simulink model "SIMU_DIF_CBF_ponto_sensor_param"  (R2025b)
settings: Solver=VariableStepAuto  StartTime=0.0  StopTime=10.0  RelTol=1e-3
undefined symbols (not defined in the file): c, l, lambda, psc, rs, theta0, thg, x0, xg, xo, y0, yg, yo
settings Model: Creator=ADM  LastModifiedBy=Dell
settings DataIOCC: ReturnWorkspaceOutputs=off

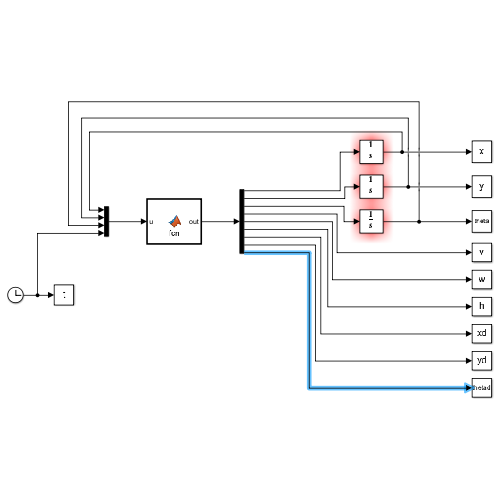
[thumbnail: Simulink's stored preview of the top-level diagram]
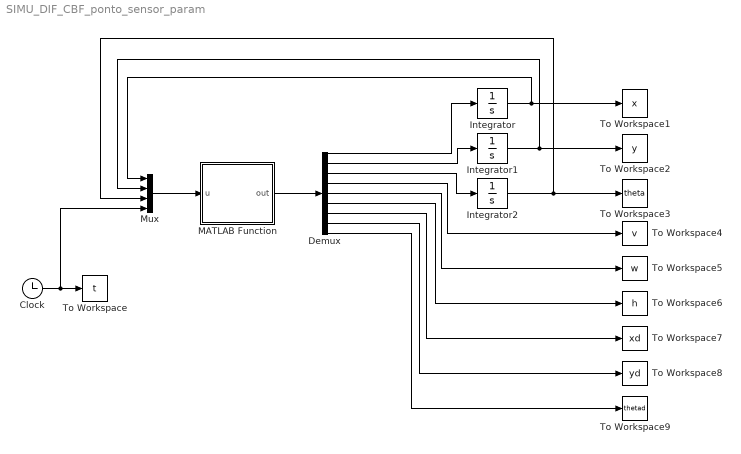
== system SIMU_DIF_CBF_ponto_sensor_param ==
  Clock : Clock
  Demux : Demux  Outputs=9
  Integrator : Integrator  InitialCondition=x0
  Integrator1 : Integrator  InitialCondition=y0
  Integrator2 : Integrator  InitialCondition=theta0
  MATLAB Function : MATLAB Function  TreatAsAtomicUnit=on
  Mux : Mux
  To Workspace : ToWorkspace  VariableName=t  SampleTime=-1
  To Workspace1 : ToWorkspace  VariableName=x  SampleTime=-1
  To Workspace2 : ToWorkspace  VariableName=y  SampleTime=-1
  To Workspace3 : ToWorkspace  VariableName=theta  SampleTime=-1
  To Workspace4 : ToWorkspace  VariableName=v  SampleTime=-1
  To Workspace5 : ToWorkspace  VariableName=w  SampleTime=-1
  To Workspace6 : ToWorkspace  VariableName=h  SampleTime=-1
  To Workspace7 : ToWorkspace  VariableName=xd  SampleTime=-1
  To Workspace8 : ToWorkspace  VariableName=yd  SampleTime=-1
  To Workspace9 : ToWorkspace  VariableName=thetad  SampleTime=-1
  wires:
  Clock/1 -> Mux/4, To Workspace/1
  Mux/1 -> MATLAB Function/1(u)
  MATLAB Function/1(out) -> Demux/1
  Demux/1 -> Integrator/1
  Demux/2 -> Integrator1/1
  Demux/3 -> Integrator2/1
  Integrator/1 -> To Workspace1/1, Mux/1
  Integrator1/1 -> To Workspace2/1, Mux/2
  Integrator2/1 -> To Workspace3/1, Mux/3
  Demux/4 -> To Workspace4/1
  Demux/5 -> To Workspace5/1
  Demux/6 -> To Workspace6/1
  Demux/7 -> To Workspace7/1
  Demux/8 -> To Workspace8/1
  Demux/9 -> To Workspace9/1

== matlab function SIMU_DIF_CBF_ponto_sensor_param/MATLAB Function ==
  data: u input size=4; out output size=9; xo parameter; yo parameter; l parameter; rs parameter; psc parameter; c parameter; lambda parameter; thg parameter; xg parameter; yg parameter
% https://chatgpt.com/c/6a83ac82-4ac8-83e9-bd58-c73133d80347
% tópico 3 - explica porque ficou pior com CLF + CBF
function out = fcn(u, xo, yo, xg, yg, thg, l, rs, psc, c, lambda)
x = u(1);
y = u(2);
theta = u(3);
t = u(4);

f_model = [0;0;0];
g_model = [cos(theta) 0;sin(theta) 0;0 1];

% % Atenção que nas referências lineares se o robô parar no centro do
% obtáculo, ele trava devido a dinâmica da CBF. Se jogar o obstáculo um pouco para baixo, ele escapa. Precisa estabeler uma
% lógica para ele escapar desta situação. Uma sugestão: forçar o robô ir para o lado ou virar.

% % Referência para pose
% xd = 5;
% yd = 5;
% thetad = pi/4;
% xd_dot = 0;
% yd_dot = 0;
% thetad_dot = 0;

% % Referência reta
% xd = 0.1*t;
% yd = 0;
% xd_dot = 0.1;
% yd_dot = 0;
% w_ref_const = 0;
% thetad = atan2(yd_dot, xd_dot);
% thetad_dot = w_ref_const;

% % Referência reta
% xd = 0.1*t;
% yd = 0.1*t;
% xd_dot = 0.1;
% yd_dot = 0.1;
% w_ref_const = 0;
% thetad = atan2(yd_dot, xd_dot);
% thetad_dot = w_ref_const;

% % % Referência de trajetória circular
% ===== OBSTACULOS (lidos do INIT) =====
obs  = [xo(:), yo(:)];
nobs = size(obs,1);

% ===== PONTO DE CHEGADA GUIADO POR "SENSOR" (sem trajetoria definida) =====
% A cada instante o robo usa sua propria pose, o ponto de chegada G e os obstaculos ao alcance.
% O alvo fica a Ld a frente, na direcao de G, deslocado lateralmente quando um obstaculo
% bloqueia o caminho direto (lado de MENOR desvio; exatamente sobre a linha: pela direita).
G    = [xg; yg];  thG = thg;    % ponto e orientacao de chegada (parametros xg, yg, thg do INIT)
m    = 0.05;    % folga alem de rs
pw   = 1.2;     % meia-largura da deformacao [m]
Ld   = 0.6;     % distancia do alvo a frente do robo [m]
Lb   = 1.5;     % distancia de G a partir da qual a orientacao final passa a contar [m]
Rsen = 3.0;     % alcance do sensor de obstaculos [m]
Lrot = 0.005;   % distancia de G a partir da qual o robo gira no lugar ate thG [m] (5 mm)
cm   = rs + m;
gx = G(1) - x;  gy = G(2) - y;
Lg = sqrt(gx^2 + gy^2);
if Lg > 1e-6
    ur = [gx; gy]/Lg;
else
    ur = [cos(theta); sin(theta)];
end
nr = [-ur(2); ur(1)];
angG = atan2(ur(2), ur(1));
st = min(Lg, Ld);
l0 = 0;  l1 = 0;
for i = 1:nobs
    so   = (obs(i,1)-x)*ur(1) + (obs(i,2)-y)*ur(2);
    dlat = (obs(i,1)-x)*nr(1) + (obs(i,2)-y)*nr(2);
    if so > -0.3 && so < min(Rsen, Lg + 0.3) && abs(dlat) < cm   % so obstaculos ao alcance e antes de G
        if abs(dlat) < 1e-3
            ell = -cm;
        else
            ell = dlat - sign(dlat)*cm;
        end
        sg = (st - so)/pw;
        if abs(sg) < 1
            l0 = l0 + ell*0.5*(1 + cos(pi*sg));
            l1 = l1 - ell*0.5*sin(pi*sg)*pi/pw;
        end
    end
end
xd = x + st*ur(1) + l0*nr(1);           % alvo
yd = y + st*ur(2) + l0*nr(2);
tht  = angG + atan(l1);                 % orientacao tangente ao desvio
lamb = min(max(1 - Lg/Lb, 0), 1);       % 0 longe de G, 1 ao chegar
thetad = tht + lamb*atan2(sin(thG - tht), cos(thG - tht));
xd_dot = 0;  yd_dot = 0;  thetad_dot = 0;

% % CLF + CBF - Vale para pose e trajetória
% % Primeira sugestão para V
% V = ((xd-x)^2 + (yd-y)^2 + (wrapToPi(thetad-theta))^2)/2;
% %V = ((xd-x)^2 + (yd-y)^2 + (thetad-theta)^2)/2;
% %V = ((x-xd)^2 + (y-yd)^2 + (theta-thetad)^2)/2;
% LfV = 0;
% LgV = [cos(theta)*(x - xd) + sin(theta)*(y - yd), wrapToPi(theta - thetad)];
% %LgV = [cos(theta)*(x - xd) + sin(theta)*(y - yd), theta - thetad];
% Vt = - thetad_dot*(wrapToPi(theta - thetad)) - xd_dot*(x - xd) - yd_dot*(y - yd);
% %Vt = - thetad_dot*(theta - thetad) - xd_dot*(x - xd) - yd_dot*(y - yd);

% % Teoricamente o mesmo resultado da CLF anterior - Só muda que não foram
% feitas as siplificações
% ex = cos(theta)*(xd-x) + sin(theta)*(yd-y);
% ey = -sin(theta)*(xd-x) + cos(theta)*(yd-y);
% etheta = wrapToPi(thetad-theta);
% % ex = cos(theta)*(x-xd) + sin(theta)*(y-yd);
% % ey = -sin(theta)*(x-xd) + cos(theta)*(y-yd);
% % etheta = wrapToPi(theta-thetad);
% V = ((ex)^2 + (ey)^2 + (etheta)^2)/2;
% % V = (wrapToPi(theta - thetad))^2/2 + (cos(theta)*(x - xd) + sin(theta)*(y - yd))^2/2 + (cos(theta)*(y - yd) - sin(theta)*(x - xd))^2/2;
% % V = (theta - thetad)^2/2 + (cos(theta)*(x - xd) + sin(theta)*(y - yd))^2/2 + (cos(theta)*(y - yd) - sin(theta)*(x - xd))^2/2;
% LfV = 0;
% %LfV = 0;
% %LgV = [cos(theta)*(cos(theta)*(cos(theta)*(x - xd) + sin(theta)*(y - yd)) - sin(theta)*(cos(theta)*(y - yd) - sin(theta)*(x - xd))) + sin(theta)*(cos(theta)*(cos(theta)*(y - yd) - sin(theta)*(x - xd)) + sin(theta)*(cos(theta)*(x - xd) + sin(theta)*(y - yd))), theta - thetad];
% %LgV = [cos(theta)*(cos(theta)*(cos(theta)*(x - xd) + sin(theta)*(y - yd)) - sin(theta)*(cos(theta)*(y - yd) - sin(theta)*(x - xd))) + sin(theta)*(cos(theta)*(cos(theta)*(y - yd) - sin(theta)*(x - xd)) + sin(theta)*(cos(theta)*(x - xd) + sin(theta)*(y - yd))), theta - thetad];
% LgV = [x*cos(theta) - xd*cos(theta) + y*sin(theta) - yd*sin(theta), wrapToPi(theta - thetad)];
% %LgV = [x*cos(theta) - xd*cos(theta) + y*sin(theta) - yd*sin(theta), theta - thetad];
% % Resposta Chatgpt
% %LgV = [cos(theta)*(x-xd) + sin(theta)*(y-yd), theta-thetad];
% % https://chatgpt.com/c/6a83ac82-4ac8-83e9-bd58-c73133d80347
% % tópico 5 e 6 explica porque usar este Vt
% %Vt = - xd_dot*(cos(theta)*(cos(theta)*(x - xd) + sin(theta)*(y - yd)) - sin(theta)*(cos(theta)*(y - yd) - sin(theta)*(x - xd))) - yd_dot*(cos(theta)*(cos(theta)*(y - yd) - sin(theta)*(x - xd)) + sin(theta)*(cos(theta)*(x - xd) + sin(theta)*(y - yd))) - thetad_dot*(theta - thetad);
% %Vt = - xd_dot*(cos(theta)*(cos(theta)*(x - xd) + sin(theta)*(y - yd)) - sin(theta)*(cos(theta)*(y - yd) - sin(theta)*(x - xd))) - yd_dot*(cos(theta)*(cos(theta)*(y - yd) - sin(theta)*(x - xd)) + sin(theta)*(cos(theta)*(x - xd) + sin(theta)*(y - yd))) - thetad_dot*(theta - thetad);
% %Vt = thetad*thetad_dot - theta*thetad_dot - x*xd_dot + xd*xd_dot - y*yd_dot + yd*yd_dot;
% %Vt = thetad*thetad_dot - theta*thetad_dot - x*xd_dot + xd*xd_dot - y*yd_dot + yd*yd_dot;
% Vt = - thetad_dot*(wrapToPi(theta - thetad)) - xd_dot*(x - xd) - yd_dot*(y - yd);

% % Outra sugestão de V - Resultados próximos
% % https://chatgpt.com/c/6ab10b65-7680-83e9-af95-79e091eac54d - explicação
% % a favor desta CLF - se for usar esta CLF, preciso descobrir de qual
% % referência o chatgpt tirou esta CLF
ex = cos(theta)*(xd-x) + sin(theta)*(yd-y);
ey = -sin(theta)*(xd-x) + cos(theta)*(yd-y);
etheta = thetad-theta;
%etheta = wrapToPi(thetad-theta);
ctheta = 1;
V = ((ex)^2 + (ey)^2)/2 + ctheta*(1-cos(etheta));
LfV = 0;
% LgV = [cos(theta)*(cos(theta)*(cos(theta)*(x - xd) + sin(theta)*(y - yd)) - sin(theta)*(cos(theta)*(y - yd) - sin(theta)*(x - xd))) + sin(theta)*(cos(theta)*(cos(theta)*(y - yd) - sin(theta)*(x - xd)) + sin(theta)*(cos(theta)*(x - xd) + sin(theta)*(y - yd))), ctheta*sin(theta - thetad)];
LgV = [x*cos(theta) - xd*cos(theta) + y*sin(theta) - yd*sin(theta), ctheta*sin(theta - thetad)];
% Vt = - xd_dot*(cos(theta)*(cos(theta)*(x - xd) + sin(theta)*(y - yd)) - sin(theta)*(cos(theta)*(y - yd) - sin(theta)*(x - xd))) - yd_dot*(cos(theta)*(cos(theta)*(y - yd) - sin(theta)*(x - xd)) + sin(theta)*(cos(theta)*(x - xd) + sin(theta)*(y - yd))) - ctheta*thetad_dot*sin(theta - thetad);
Vt = xd*xd_dot - x*xd_dot - y*yd_dot + yd*yd_dot - ctheta*thetad_dot*sin(theta - thetad);

% % CBF
% ===== OBSTACULOS (CBF individual + vies de lado) =====
% ===== OBSTACULOS: vetores xo, yo vindos do INIT (um elemento por obstaculo) =====
side = 1;      % +1 desvia virando a esquerda, -1 a direita
hact = 1.0;    % h abaixo do qual o vies de lado comeca
wb   = 0.0;    % intensidade maxima do vies em w [rad/s]

px = x + l*cos(theta);
py = y + l*sin(theta);

hv    = zeros(nobs,1);
Lghm  = zeros(nobs,2);
wbias = 0;
for i = 1:nobs
    dx = px - obs(i,1);
    dy = py - obs(i,2);
    hv(i)     = dx^2 + dy^2 - rs^2;
    Lghm(i,:) = [2*dx*cos(theta) + 2*dy*sin(theta), ...
                 2*l*(dy*cos(theta) - dx*sin(theta))];
    dist  = max(sqrt(dx^2 + dy^2), 1e-6);
    a     = max(0, min(1, 1 - hv(i)/hact));
    ahead = max(0, (-dx*cos(theta) - dy*sin(theta))/dist);
    wbias = wbias + side*a*ahead;
end
wbias = wb*max(-1, min(1, wbias));

h   = min(hv);   % apenas para o grafico
Lfh = 0;

% ===== CONTROLE NOMINAL DE RASTREAMENTO (Kanayama) =====
kp = 0.8;  ka = 2.0;  kb = -0.5;  krot = 2.0;   % controlador polar (kp>0, kb<0, ka>kp)
rho = sqrt((xd-x)^2 + (yd-y)^2);
al  = atan2(yd-y, xd-x) - theta;
al  = atan2(sin(al), cos(al));
be  = thetad - theta - al;
be  = atan2(sin(be), cos(be));
v_nom = kp*rho*max(cos(al), 0);         % nao anda de re: vira antes de avancar
w_nom = ka*al + kb*lamb*be + wbias;
if Lg < Lrot                            % chegou: gira no lugar ate a orientacao final
    v_nom = 0;
    w_nom = krot*atan2(sin(thG - theta), cos(thG - theta));
end
u_nom = [v_nom; w_nom];

% QP: minimiza ||u - u_nom||^2 + psc*delta^2
Hqp = [1 0 0; 0 1 0; 0 0 psc];
Fqp = [-u_nom; 0];

% ===== RESTRICOES: 1 CLF + nobs CBFs + limites de v e w =====
Aqp = zeros(nobs+5,3);
bqp = zeros(nobs+5,1);
Aqp(1,:) = [LgV, -1];
bqp(1)   = -LfV - c*V - Vt;
for i = 1:nobs
    Aqp(1+i,:) = [-Lghm(i,:), 0];
    bqp(1+i)   = Lfh + lambda*hv(i);
end
Aqp(nobs+2:nobs+5,:) = [1 0 0; -1 0 0; 0 1 0; 0 -1 0];
bqp(nobs+2:nobs+5)   = 2;

ucont = [0;0;0];
coder.extrinsic('QPhild');
ucont = QPhild(Hqp,Fqp,Aqp,bqp);
uc = [ucont(1,1);ucont(2,1)];
xmponto = f_model + g_model*uc;

% Saidas de referencia para o grafico: CIRCULO ORIGINAL (sem deformacao).
% O controle usa internamente a referencia deformada (xd, yd, thetad).
% Saidas de referencia para o grafico: ponto de chegada.
xd0 = G(1);
yd0 = G(2);
thetad0 = thG;
out = [xmponto(1,1);xmponto(2,1);xmponto(3,1);uc(1,1);uc(2,1);h;xd0;yd0;thetad0];








% % % Controle nominal + CBF - Safety Filter
% function out = fcn(u, xo, yo, l, rs, psc, c, lambda)
% x = u(1);
% y = u(2);
% theta = u(3);
% t = u(4);
% 
% f_model = [0;0;0];
% g_model = [cos(theta) 0;sin(theta) 0;0 1];
% 
% % % % Atenção que nas referências lineares se o robô parar no centro do
% % % obtáculo, ele trava devido a dinâmica da CBF. Se jogar o obstáculo um pouco para baixo, ele escapa 
% % % (Para o controle nominal, precisa jogar mais para baixo ainda). Precisa estabeler uma
% % % lógica para ele escapar desta situação. Uma sugestão: forçar o robô ir para o lado ou virar.
% 
% % % % Referência reta
% % xd = 0.1*t;
% % yd = 0;
% % xd_dot = 0.1;
% % yd_dot = 0;
% % w_ref_const = 0;
% % vd = sqrt(xd_dot^2 + yd_dot^2);
% % thetad = atan2(yd_dot, xd_dot);
% % wd = w_ref_const;
% 
% % % % Referência reta
% % xd = 0.1*t;
% % yd = 0.1*t;
% % xd_dot = 0.1;
% % yd_dot = 0.1;
% % w_ref_const = 0;
% % vd = sqrt(xd_dot^2 + yd_dot^2);
% % thetad = atan2(yd_dot, xd_dot);
% % wd = w_ref_const;
% 
% % % % Referência de trajetória circular
% % R = 2;
% % w_ref_const = 0.25;
% % xd = R*cos(w_ref_const*t);
% % yd = R*sin(w_ref_const*t);
% % xd_dot = -R*w_ref_const*sin(w_ref_const*t);
% % yd_dot =  R*w_ref_const*cos(w_ref_const*t);
% % vd = sqrt(xd_dot^2 + yd_dot^2);
% % thetad = atan2(yd_dot, xd_dot);
% % wd = w_ref_const;
% 
% % % % Controlador nominal para trajetória
% % kx = 1.5;
% % ky = 3.0;
% % ktheta = 2.0;
% % ex = cos(theta)*(xd-x) + sin(theta)*(yd-y);
% % ey = -sin(theta)*(xd-x) + cos(theta)*(yd-y);
% % %etheta = thetad-theta;
% % etheta = wrapToPi(thetad-theta);
% % % % https://chatgpt.com/c/6a83ac82-4ac8-83e9-bd58-c73133d80347 - nos
% % % % tópicos finais explica que com ky*vd*ey é melhor - nas simulações também
% % unom = [vd*cos(etheta)+kx*ex;wd+ky*vd*ey+ktheta*sin(etheta)];
% % %unom = [vd*cos(etheta)+kx*ex;wd+ky*ey+ktheta*sin(etheta)];
% 
% % % % Referência para pose
% xd = 5;
% yd = 5;
% thetad = pi/4;
% xd_dot = 0;
% yd_dot = 0;
% thetad_dot = 0;
% 
% % % % Controlador nominal para pose
% ex = xd - x;
% ey = yd - y;
% pho = sqrt(ex^2 + ey^2);
% alfa = atan2(ey,ex) - theta;
% % % wrapToPi e atan2 tem a mesma função: garantir que o ângulo fique entre
% % -pi e + pi
% %alfa = atan2(sin(alfa),cos(alfa));
% alfa = wrapToPi(alfa);
% % testar com estas duas possibilidades para beta
% %beta = thetad - theta;
% beta = thetad - theta - alfa;
% % % wrapToPi e atan2 tem a mesma função: garantir que o ângulo fique entre
% % -pi e + pi
% beta = wrapToPi(beta);
% % beta = atan2(sin(beta),cos(beta));
% kpho = 0.5;
% kalfa = 2;
% %kbeta = 0.5;
% kbeta = -0.5;
% % Tem duas opções de controle:
% % a princípio os resultados são parecidos, mas a primeira opção é melhor
% unom = [kpho*pho*cos(alfa);kalfa*alfa + kbeta*beta];
% % kv = 0.5;
% % kw = 1.0;
% % unom = [kv*pho;kw*alfa];
% 
% % ex = cos(theta)*(xd-x) + sin(theta)*(yd-y);
% % ey = -sin(theta)*(xd-x) + cos(theta)*(yd-y);
% % etheta = thetad-theta;
% % etheta = atan2(sin(etheta),cos(etheta));
% % kx = 5;
% % ky = 5;
% % ktheta = 5;
% % unom = [kx*ex;ky*ey + ktheta*etheta];
% 
% % % CBF
% h = (x+l*cos(theta)-xo)^2 + (y+l*sin(theta)-yo)^2 - (rs)^2;
% Lfh = 0;
% Lgh = [sin(theta)*(2*y - 2*yo + 2*l*sin(theta)) + cos(theta)*(2*x - 2*xo + 2*l*cos(theta)), 2*l*cos(theta)*(y - yo + l*sin(theta)) - 2*l*sin(theta)*(x - xo + l*cos(theta))];
% %Lgh = [sin(theta)*(2*y - 2*yo + 2*l*sin(theta)) + cos(theta)*(2*x - 2*xo + 2*l*cos(theta)), 2*l*cos(theta)*(y - yo + l*sin(theta)) - 2*l*sin(theta)*(x - xo + l*cos(theta))];
% 
% % % Controlador Final
% Hqp = [2];
% Fqp = [-2*unom];
% % Aqp = [-Lgh];
% % bqp = [Lfh+lambda*h];
% Aqp = [-Lgh;1 0;-1 0;0 1;0 -1];
% bqp = [Lfh+lambda*h;0.5;0.5;1.5;1.5];
% uc = [0;0];
% coder.extrinsic('QPhild');
% uc = QPhild(Hqp,Fqp,Aqp,bqp);
% xmponto = f_model + g_model*uc;
% %xmponto = f_model + g_model*unom;
% 
% % % Soluções Fechadas
% % % Não sei porque esta solução não funciona para este problema
% % %uc = [0;0];
% % I = Lfh + Lgh*unom;
% % J = lambda*h;
% % if (I<J)
% % ucont = -((I-J)/(norm(Lgh))^2)*(transpose(Lgh));
% % %ucont = -((I-J)/(norm(Lgh))*(norm(Lgh)))*transpose(Lgh);
% % %ucont = -((I-J)/(Lgh*transpose(Lgh)))*(transpose(Lgh));
% % else
% % ucont = [0;0];
% % end
% % uc = ucont+unom;
% % if uc(1,1)>=0.5
% % uc(1,1)=0.5;  
% % end
% % if uc(1,1)<=-0.5
% % uc(1,1)=-0.5;  
% % end
% % if uc(2,1)>=1.5
% % uc(2,1)=1.5;  
% % end
% % if uc(2,1)<=-1.5
% % uc(2,1)=-1.5;  
% % end
% % xmponto = f_model + g_model*uc;
% % %xmponto = f_model + g_model*unom;
% 
% % uc = [0;0];
% % I = LfB + LgB*unom;
% % J = lambda*B;
% % if (I>J)
% % ucont = -((I-J)/(norm(LgB))^2)*transpose(LgB);
% % else
% % ucont = [0;0];
% % end
% % uc = ucont+unom;
% % xmponto = f_model + g_model*(uc);
% % %xmponto = f_model + g_model*unom;
% % 
% % 
% % % Esta solução funciona
% % % uc = [0;0];
% % phi = Lfh + Lgh*unom + lambda*h;
% % if (phi<0)
% % uc = unom - (phi*transpose(Lgh))/(Lgh*transpose(Lgh));
% % else
% % uc = unom - [0;0];
% % end
% % if uc(1,1)>=0.5
% % uc(1,1)=0.5;  
% % end
% % if uc(1,1)<=-0.5
% % uc(1,1)=-0.5;  
% % end
% % if uc(2,1)>=1.5
% % uc(2,1)=1.5;  
% % end
% % if uc(2,1)<=-1.5
% % uc(2,1)=-1.5;  
% % end
% % xmponto = f_model + g_model*uc;
% % %xmponto = f_model + g_model*unom;
% 
% out = [xmponto(1,1);xmponto(2,1);xmponto(3,1);uc(1,1);uc(2,1);h;xd;yd;thetad];
